simulink model "sm_ratchet_pawl"  (R2025a)
settings: Solver=daessc  StartTime=0.0  StopTime=30  MaxStep=0.01  RelTol=1e-3  AbsTol=1e-3  EnableMultiTasking=on
PreLoadFcn:
  | sm_ratchet_pawl_param
undefined symbols (not defined in the file): A, B, C, D, F, pawl_driver, pawl_locking, ratchet_arm, ratchet_wheel, X, Y, Z
libraries: sm_lib x20, sm_ratchet_pawl_lib x18, nesl_utility x4, fl_lib x3
CloseFcn:
  | try,close(h1_sm_ratchet_pawl),end
  | clear h1_sm_ratchet_pawl
  | try,close(h2_sm_ratchet_pawl),end
  | clear h2_sm_ratchet_pawl
  | try,close(h3_sm_ratchet_pawl),end
  | clear h3_sm_ratchet_pawl
  | try,close(h4_sm_ratchet_pawl),end
  | clear h4_sm_ratchet_pawl
  | 
  | try,close(h1_Extr_Data_Pawl),end
  | try,close(h1_Extr_Data_Ratchet_Wheel),end
Description:
  | Copyright 2024-2026 The MathWorks, Inc.
settings Model: Creator=smiller  LastModifiedBy=smiller
settings SolverCC: AutoScaleAbsTol=off  AlgebraicLoopSolver=TrustRegion  MaxZcPerStep=1.0
settings DataIOCC: LimitDataPoints=on  MaxDataPoints=10000  ReturnWorkspaceOutputs=off  SignalLoggingName=logsout_sm_ratchet_pawl
settings OptimizationCC: ReuseModelBlockBuffer=off  LifeSpan=inf
settings DebuggingCC: UnconnectedInputMsg=warning  UnconnectedOutputMsg=warning  UnconnectedLineMsg=warning  AllowSymbolicDim=off  SubsystemReferenceDiagnosticForUnitTest=warning  SFUnexpectedBacktrackingDiag=warning  SFNoUnconditionalDefaultTransitionDiag=warning  SFExecutionAtInitializationDiag=none  ArithmeticOperatorsInVariantConditions=warning
settings ModelReferenceCC: EnableRefExpFcnMdlSchedulingChecks=on
settings SFSimCC: SimUseLocalCustomCode=off  CustomCodeUndefinedFunction=UseInterfaceOnly
settings RTWCC: RTWUseLocalCustomCode=off  GPUComputeCapability=3.5  DLArmComputeVersion=19.05
settings CodeAppCC: StateflowObjectComments=on
settings GRTTargetCC: TargetLangStandard=C89/C90 (ANSI)
settings ConfigComp: CovMetricSettings=dw  CovSaveCumulativeToWorkspaceVar=on  CovSaveSingleToWorkspaceVar=on  CovExternalEMLEnable=off  CovSFcnEnable=off
settings SimscapeCC: SimscapeLogType=all  SimscapeLogSimulationStatistics=on  SimscapeLogName=simlog_sm_ratchet_pawl  SimscapeLogDataHistory=100000.0
settings ExplorerConfigSet: InternalSimMechanicsExplorerSettings="<ExplorerConfiguration><canonicalview>default</canonicalview><AnimationSetting><BasePlaybackSpeed>1.0</BasePlaybackSpeed><PlaybackSpeedFactor>2.0</PlaybackSpeedFactor></AnimationSetting><TilePanel><TileInfo><Tiles Columns=\"2\" Count=\"3\" Rows=\"2\"><Column Weight=\"0.6446\"/><Column Weight=\"0.3554\"/><Row Weight=\"0.4352\"/><Row Weight=\"0.5648\"/><Tile Height=\"2\" Width=\"1\" X=\"0\" Y=\"0\"/><Tile Height=\"1\" Width=\"1\" X=\"1\" Y=\"0\"/><Tile Height=\"1\" Width=\"1\" X=\"1\" Y=\"1\"/></Tiles></TileInfo><SceneInfo><SceneViewer><BGColor><R>1</R><G>1</G><B>1</B></BGColor><Camera><DoPerspective>off</DoPerspective><Position><X>0.0514746329653971782</X><Y>0.0112521347858783351</Y><Z>0.995249982152964785</Z></Position><Center><X>0.0514746329653971782</X><Y>0.0112521347858783351</Y><Z>-0.00475001784703521501</Z></Center><Up><X>0</X><Y>1</Y><Z>-0</Z></Up><ViewLimDist>1</ViewLimDist><YLim>0.117248588338494303</YLim><XLim>0.158994678564636227</XLim></Camera></SceneViewer><SceneViewer><BGColor><R>1</R><G>1</G><B>1</B></BGColor><Camera><DoPerspective>off</DoPerspective><Position><X>-0.560100967125156224</X><Y>0.346484843060087866</Y><Z>0.771615368247267508</Z></Position><Center><X>-0.00343975445121295865</X><Y>0.095498245923905864</Y><Z>-0.0203025709120879597</Z></Center><Up><X>0.214451241288348721</X><Y>0.964373692155350071</Y><Z>-0.154900119394868807</Z></Up><ViewLimDist>1</ViewLimDist><YLim>0.0292488636148055016</YLim><XLim>0.0509233203174103768</XLim></Camera></SceneViewer><SceneViewer><BGColor><R>1</R><G>1</G><B>1</B></BGColor><Camera><DoPerspective>off</DoPerspective><Position><X>0.849936568602107645</X><Y>0.00451951510809854573</Y><Z>0.588389331993768971</Z></Position><Center><X>0.0650124134104529405</X><Y>0.0227163583315792908</Y><Z>-0.0309352561612741273</Z></Center><Up><X>0.0909807338167105406</X><Y>0.992118625029582368</Y><Z>-0.0861576458800011047</Z></Up><ViewLimDist>1</ViewLimDist><YLim>0.0639705507090228137</YLim><XLim>0.0854896962074708638</XLim></Camera></SceneViewer></SceneInfo></TilePanel><MechEditorPanel><Cameras/><GfxPanelCameraMap/><VideoCreator><PlaybackSpeedRatio>2</PlaybackSpeedRatio><FrameRate>30</FrameRate><VideoFormat>MPEG-4</VideoFormat><FrameSize>auto</FrameSize></VideoCreator></MechEditorPanel></ExplorerConfiguration>"

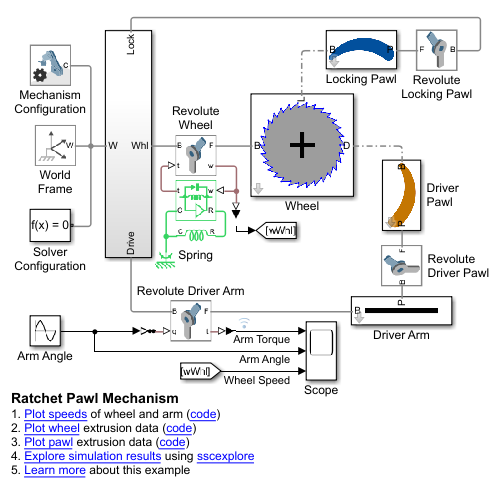
[thumbnail: Simulink's stored preview of the top-level diagram]
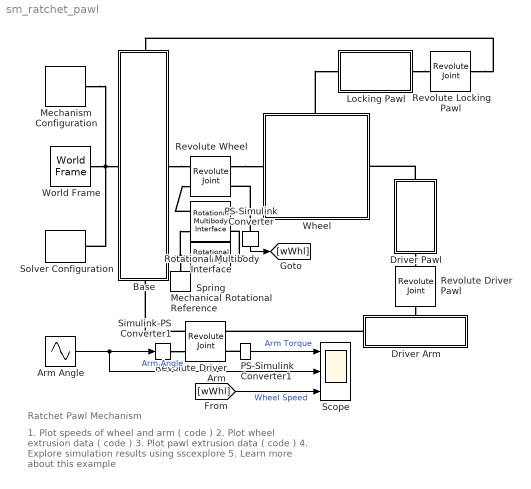
== system sm_ratchet_pawl ==
  note: Ratchet Pawl Mechanism
  note: 1. Plot speeds of wheel and arm ( code )
      | 2. Plot wheel extrusion data ( code )
      | 3. Plot pawl extrusion data ( code )
      | 4. Explore simulation results using sscexplore
      | 5. Learn more about this example
  Arm Angle : Sin  Amplitude=30  Frequency=2*pi/5  SampleTime=0
  Base : Subsystem
      settings: PortSchema="{\"entries\":[{\"content\":{\"sides\":[{\"content\":{\"connectorIds\":[\"LConn1\"]},\"type\":\"ConnectorPlacement.EquallySpacedRectSide\",\"uuid\":\"b6069478-d7cb-4b03-b34f-7e279460368d\"},{\"content\":{\"connectorIds\":[\"RConn1\"],\"side\":\"RIGHT\"},\"type\":\"ConnectorPlacement.EquallySpacedRectSide\",\"uuid\":\"d4387135-640e-415f-ac36-e6f51d44e49d\"},{\"content\":{\"connectorIds\":[\"LConn2\"],\"side\":\"TOP\"},\"type\":\"ConnectorPlacement.EquallySpacedRectSide\",\"uuid\":\"9397bae0-a413-4c70-a9df-3b58371f95bd\"},{\"content\":{\"connectorIds\":[\"RConn2\"],\"side\":\"BOTTOM\"},\"type\":\"ConnectorPlacement.EquallySpacedRectSide\",\"uuid\":\"bb7f362f-dbc7-4f0c-a5eb-cae814777abd\"}]},\"type\":\"ConnectorPlacement.EquallySpacedConnector\",\"uuid\":\"025a31d6-c78e-4390-922c-78c8ee846b7b\"}],\"packageUris\":[\"http://schema.mathworks.com/mf0/Connector/R2020b\"],\"version\":\"1.0\"}"
  Driver Pawl : Subsystem
      mask Display: image('sm_ratchet_pawl_driver_pawl.png');
  Driver Arm : Subsystem
      settings: PortSchema="{\"entries\":[{\"content\":{\"sides\":[{\"content\":{},\"type\":\"ConnectorPlacement.EquallySpacedRectSide\",\"uuid\":\"931ad4cf-5a99-4c9c-9c4c-5cc9ae808209\"},{\"content\":{\"connectorIds\":[\"RConn1\"],\"side\":\"RIGHT\"},\"type\":\"ConnectorPlacement.EquallySpacedRectSide\",\"uuid\":\"6aeb9602-858e-433f-b8ee-b1fa4efa2662\"},{\"content\":{\"connectorIds\":[\"LConn1\"],\"side\":\"TOP\"},\"type\":\"ConnectorPlacement.EquallySpacedRectSide\",\"uuid\":\"8a68191e-bbb5-4d51-a354-3893ab4bb353\"}]},\"type\":\"ConnectorPlacement.EquallySpacedConnector\",\"uuid\":\"f1c0db8b-851d-448f-812d-c20024300439\"}],\"packageUris\":[\"http://schema.mathworks.com/mf0/Connector/R2020b\"],\"version\":\"1.0\"}"
      mask Display: image('sm_ratchet_pawl_driver_arm.png');
  Locking Pawl : Subsystem
      mask Display: image('sm_ratchet_pawl_locking_pawl.png')
  Mechanical Rotational Reference : fl_lib/Mechanical/Rotational Elements/Mechanical Rotational Reference
  Mechanism Configuration : sm_lib/Utilities/Mechanism Configuration  UniformGravity=Constant  GravityVector=[0 0 -9.80665]  GravityVectorUnits=m/s^2  LinearizationDelta=0.001  JointModeTransitionNonlinearIterations=2
  PS-Simulink Converter : nesl_utility/PS-Simulink Converter  PhysicalDomain=network_engine_domain  SubClassName=ps_output  LeftPortType=input  RightPortType=output  PseudoPeriodic=off  Frequencies=[]  VectorFormat=inherit  Unit=inherit  AffineConversion=off
  PS-Simulink Converter1 : nesl_utility/PS-Simulink Converter  PhysicalDomain=network_engine_domain  SubClassName=ps_output  LeftPortType=input  RightPortType=output  PseudoPeriodic=off  Frequencies=[]  VectorFormat=inherit  Unit=1  AffineConversion=off
  Revolute Driver Pawl : sm_lib/Joints/Revolute Joint  JointMode=Normal  CompositeWrenchDir=FollowerOnBase  CompositeWrenchFrame=BaseFrame  SenseConstraintForce=off  SenseConstraintTorque=off  SenseTotalForce=off  SenseTotalTorque=off  PositionTargetSpecify=on  PositionTargetPriority=High  PositionTargetValue=0  PositionTargetValueUnits=deg  VelocityTargetSpecify=off  VelocityTargetPriority=High  VelocityTargetValue=0  VelocityTargetValueUnits=deg/s  EquilibriumPosition=30  EquilibriumPositionUnits=deg  SpringStiffness=0.1  SpringStiffnessUnits=N*m/deg  DampingCoefficient=0.02  DampingCoefficientUnits=N*m/(deg/s)  LowerLimitSpecify=off  LowerLimitBound=-90  LowerLimitBoundUnits=deg  LowerLimitStiffness=1e4  LowerLimitStiffnessUnits=N*m/deg  LowerLimitDamping=10  LowerLimitDampingUnits=N*m/(deg/s)  LowerLimitTransitionRegionWidth=0.1  LowerLimitTransitionRegionWidthUnits=deg  UpperLimitSpecify=off  UpperLimitBound=90  UpperLimitBoundUnits=deg  UpperLimitStiffness=1e4  UpperLimitStiffnessUnits=N*m/deg  UpperLimitDamping=10  UpperLimitDampingUnits=N*m/(deg/s)  UpperLimitTransitionRegionWidth=0.1  UpperLimitTransitionRegionWidthUnits=deg  TorqueActuationMode=NoTorque  MotionActuationMode=ComputedMotion  SensePosition=off  SenseVelocity=off  SenseAcceleration=off  SenseTorqueForce=off  SenseLowerLimitTorqueForce=off  SenseUpperLimitTorqueForce=off
  Revolute Locking Pawl : sm_lib/Joints/Revolute Joint  JointMode=Normal  CompositeWrenchDir=FollowerOnBase  CompositeWrenchFrame=BaseFrame  SenseConstraintForce=off  SenseConstraintTorque=off  SenseTotalForce=off  SenseTotalTorque=off  PositionTargetSpecify=on  PositionTargetPriority=High  PositionTargetValue=90  PositionTargetValueUnits=deg  VelocityTargetSpecify=off  VelocityTargetPriority=High  VelocityTargetValue=0  VelocityTargetValueUnits=deg/s  EquilibriumPosition=110  EquilibriumPositionUnits=deg  SpringStiffness=0.1  SpringStiffnessUnits=N*m/deg  DampingCoefficient=0.02  DampingCoefficientUnits=N*m/(deg/s)  LowerLimitSpecify=off  LowerLimitBound=-90  LowerLimitBoundUnits=deg  LowerLimitStiffness=1e4  LowerLimitStiffnessUnits=N*m/deg  LowerLimitDamping=10  LowerLimitDampingUnits=N*m/(deg/s)  LowerLimitTransitionRegionWidth=0.1  LowerLimitTransitionRegionWidthUnits=deg  UpperLimitSpecify=off  UpperLimitBound=90  UpperLimitBoundUnits=deg  UpperLimitStiffness=1e4  UpperLimitStiffnessUnits=N*m/deg  UpperLimitDamping=10  UpperLimitDampingUnits=N*m/(deg/s)  UpperLimitTransitionRegionWidth=0.1  UpperLimitTransitionRegionWidthUnits=deg  TorqueActuationMode=NoTorque  MotionActuationMode=ComputedMotion  SensePosition=off  SenseVelocity=off  SenseAcceleration=off  SenseTorqueForce=off  SenseLowerLimitTorqueForce=off  SenseUpperLimitTorqueForce=off
  Revolute Wheel : sm_lib/Joints/Revolute Joint  JointMode=Normal  CompositeWrenchDir=FollowerOnBase  CompositeWrenchFrame=BaseFrame  SenseConstraintForce=off  SenseConstraintTorque=off  SenseTotalForce=off  SenseTotalTorque=off  PositionTargetSpecify=off  PositionTargetPriority=High  PositionTargetValue=0  PositionTargetValueUnits=deg  VelocityTargetSpecify=off  VelocityTargetPriority=High  VelocityTargetValue=0  VelocityTargetValueUnits=deg/s  EquilibriumPosition=0  EquilibriumPositionUnits=deg  SpringStiffness=0  SpringStiffnessUnits=N*m/deg  DampingCoefficient=0.1  DampingCoefficientUnits=N*m/(deg/s)  LowerLimitSpecify=off  LowerLimitBound=-90  LowerLimitBoundUnits=deg  LowerLimitStiffness=1e4  LowerLimitStiffnessUnits=N*m/deg  LowerLimitDamping=10  LowerLimitDampingUnits=N*m/(deg/s)  LowerLimitTransitionRegionWidth=0.1  LowerLimitTransitionRegionWidthUnits=deg  UpperLimitSpecify=off  UpperLimitBound=90  UpperLimitBoundUnits=deg  UpperLimitStiffness=1e4  UpperLimitStiffnessUnits=N*m/deg  UpperLimitDamping=10  UpperLimitDampingUnits=N*m/(deg/s)  UpperLimitTransitionRegionWidth=0.1  UpperLimitTransitionRegionWidthUnits=deg  TorqueActuationMode=InputTorque  MotionActuationMode=ComputedMotion  SensePosition=off  SenseVelocity=on  SenseAcceleration=off  SenseTorqueForce=off  SenseLowerLimitTorqueForce=off  SenseUpperLimitTorqueForce=off
  Revolute Driver Arm : sm_lib/Joints/Revolute Joint  JointMode=Normal  CompositeWrenchDir=FollowerOnBase  CompositeWrenchFrame=BaseFrame  SenseConstraintForce=off  SenseConstraintTorque=off  SenseTotalForce=off  SenseTotalTorque=off  PositionTargetSpecify=off  PositionTargetPriority=High  PositionTargetValue=0  PositionTargetValueUnits=deg  VelocityTargetSpecify=off  VelocityTargetPriority=High  VelocityTargetValue=0  VelocityTargetValueUnits=deg/s  EquilibriumPosition=0  EquilibriumPositionUnits=deg  SpringStiffness=0  SpringStiffnessUnits=N*m/deg  DampingCoefficient=0  DampingCoefficientUnits=N*m/(deg/s)  LowerLimitSpecify=off  LowerLimitBound=-90  LowerLimitBoundUnits=deg  LowerLimitStiffness=1e4  LowerLimitStiffnessUnits=N*m/deg  LowerLimitDamping=10  LowerLimitDampingUnits=N*m/(deg/s)  LowerLimitTransitionRegionWidth=0.1  LowerLimitTransitionRegionWidthUnits=deg  UpperLimitSpecify=off  UpperLimitBound=90  UpperLimitBoundUnits=deg  UpperLimitStiffness=1e4  UpperLimitStiffnessUnits=N*m/deg  UpperLimitDamping=10  UpperLimitDampingUnits=N*m/(deg/s)  UpperLimitTransitionRegionWidth=0.1  UpperLimitTransitionRegionWidthUnits=deg  TorqueActuationMode=ComputedTorque  MotionActuationMode=InputMotion  SensePosition=off  SenseVelocity=off  SenseAcceleration=off  SenseTorqueForce=on  SenseLowerLimitTorqueForce=off  SenseUpperLimitTorqueForce=off
  Rotational Multibody Interface : fl_lib/Mechanical/Multibody Interfaces/Rotational Multibody Interface
  Scope : Scope  NumInputPorts=3
      settings: ActiveDisplayYMinimum=-11.66487  ActiveDisplayYMaximum=46.52781
  Simulink-PS Converter1 : nesl_utility/Simulink-PS Converter  PhysicalDomain=network_engine_domain  SubClassName=ps_input  LeftPortType=input  RightPortType=output  PseudoPeriodic=off  Frequencies=[]  NoiseDistribution=none  NoiseParameters=[]  Unit=deg  AffineConversion=off  FilteringAndDerivatives=filter  SimscapeFilterOrder=2  InputFilterTimeConstant=0.1  UdotUserProvided=0
  Solver Configuration : nesl_utility/Solver Configuration  PhysicalDomain=network_engine_domain  SubClassName=solver  LeftPortType=input  RightPortType=generic  Tones=[]  Harmonics=[]  SimulateNoise=off  Profile=off  UseLocalSampling=off  EnableSwitchedLinearOptims=on  FrequencyDomain=off  UseCCode=off  RelTol=0.001  AbsTol=1e-06  MinStep=1e-09  ToWorkspace=off  RevertToSquareIcSolve=off  NumHomotopyIterations=100  PhasorMode=off  PhasorModeNumHarmonics=1  ConsistencySolver=NEWTON_XTOL_AFTER_FTOL  IndexReductionMethod=DerivativeReplacement  DoDC=off  ResidualTolerance=1e-09  ConsistencyTolSource=GLOBAL  ConsistencyAbsTol=0.001  ConsistencyRelTol=0.001  ConsistencyTolFactor=0.001  UseLocalSolver=off  LocalSolverChoice=NE_BACKWARD_EULER_ADVANCER  ResolveIndetEquations=on  FunctionEvalNumThread=1  LocalSolverSampleTime=0.001  DoFixedCost=off  MaxNonlinIter=3  MaxModeIter=2  ComputeImpulses=off  ImpulseIterations=2  LinearAlgebra=Sparse  LinearAlgebraNumThread=0  EquationFormulation=NE_TIME_EF  DelaysMemoryBudget=1024  AutomaticFiltering=on  FilteringTimeConstant=0.001  PartitionStorageMethod=AS_NEEDED  PartitionMemoryBudget=1024  PartitionMethod=FAST  MultibodyUseLocalSolver=off  MultibodyLocalSolverChoice=ODE1  MultibodyLocalSolverSampleTime=0.001
  Spring : fl_lib/Mechanical/Rotational Elements/Rotational Spring  spr_rate=10 N*m/rad  w_specify=off  w_priority=None  w=0 rad/s  w_nominal_specify=off  w_nominal_value=1  w_nominal_unit=rad/s  t_specify=off  t_priority=None  t=0 N*m  t_nominal_specify=off  t_nominal_value=1  t_nominal_unit=N*m  phi_specify=off  phi_priority=High  phi=0 rad  phi_nominal_specify=off  phi_nominal_value=1  phi_nominal_unit=rad
  Wheel : Subsystem
      settings: PortSchema="{\"entries\":[{\"content\":{\"sides\":[{\"content\":{\"connectorIds\":[\"LConn1\"]},\"type\":\"ConnectorPlacement.EquallySpacedRectSide\",\"uuid\":\"04441881-9c30-4d5d-be6a-59ca06764360\"},{\"content\":{\"connectorIds\":[\"RConn1\"],\"side\":\"RIGHT\"},\"type\":\"ConnectorPlacement.EquallySpacedRectSide\",\"uuid\":\"fa22e8ef-2b3e-4a8e-b49c-1688172feace\"},{\"content\":{\"connectorIds\":[\"LConn2\"],\"side\":\"TOP\"},\"type\":\"ConnectorPlacement.EquallySpacedRectSide\",\"uuid\":\"207ec217-ed21-440a-9842-994c4e25d04a\"}]},\"type\":\"ConnectorPlacement.EquallySpacedConnector\",\"uuid\":\"e84f3840-6153-4aef-b387-4bc57ec5edf1\"}],\"packageUris\":[\"http://schema.mathworks.com/mf0/Connector/R2020b\"],\"version\":\"1.0\"}"
      mask Display: image('sm_ratchet_pawl_wheel_lines.png')
  World Frame : sm_lib/Frames and Transforms/World Frame
  wires:
  [wWhl] -> Scope/3  "Wheel Speed"
  Arm Angle/1 -> Simulink-PS Converter1/1, Scope/2  "Arm Angle"
  PS-Simulink Converter1/1 -> Scope/1  "Arm Torque"
  PS-Simulink Converter/1 -> [wWhl]
  connections:
  World Frame/RConn1 -- Solver Configuration/RConn1 -- Base/LConn1 -- Mechanism Configuration/RConn1
  Driver Arm/RConn1 -- Revolute Driver Arm/RConn1
  Revolute Driver Pawl/LConn1 -- Driver Arm/LConn1
  Driver Pawl/RConn1 -- Revolute Driver Pawl/RConn1
  Revolute Wheel/RConn1 -- Wheel/LConn1
  Driver Pawl/LConn1 -- Wheel/RConn1
  Locking Pawl/RConn1 -- Revolute Locking Pawl/RConn1
  Wheel/LConn2 -- Locking Pawl/LConn1
  Simulink-PS Converter1/RConn1 -- Revolute Driver Arm/LConn2
  Revolute Locking Pawl/LConn1 -- Base/LConn2
  Revolute Driver Arm/LConn1 -- Base/RConn2
  Base/RConn1 -- Revolute Wheel/LConn1
  PS-Simulink Converter1/LConn1 -- Revolute Driver Arm/RConn2
  PS-Simulink Converter/LConn1 -- Rotational Multibody Interface/RConn1 -- Revolute Wheel/RConn2
  Rotational Multibody Interface/LConn1 -- Revolute Wheel/LConn2
  Spring/LConn1 -- Rotational Multibody Interface/RConn2
  Spring/RConn1 -- Mechanical Rotational Reference/LConn1 -- Rotational Multibody Interface/LConn2

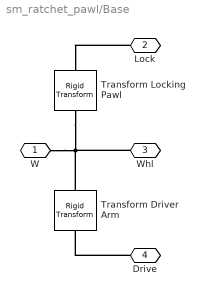
== system sm_ratchet_pawl/Base ==
  Transform Driver Arm : sm_lib/Frames and Transforms/Rigid Transform  RotationMethod=None  FollAlignAxisA=+X  BaseAlignAxisA=+Y  FollAlignAxisB=+Y  BaseAlignAxisB=+Z  RotationStandardAxis=+Z  RotationAngle=0.0  RotationAngleUnits=deg  RotationArbitraryAxis=[0 0 1]  RotationSequenceAxes=FollowerAxes  RotationSequence=XYX  RotationSequenceAngles=[0 0 0]  RotationSequenceAnglesUnits=deg  RotationMatrix=[1 0 0; 0 1 0; 0 0 1]  Quaternion=[1 0 0 0]  TranslationMethod=StandardAxis  TranslationCartesianOffset=[0 0 0]  TranslationCartesianOffsetUnits=m  TranslationStandardAxis=+Z  TranslationStandardOffset=-(ratchet_arm.depth+ratchet_wheel.depth)/2  TranslationStandardOffsetUnits=m  TranslationROffset=0  TranslationROffsetUnits=m  TranslationThetaOffset=0  TranslationThetaOffsetUnits=deg  TranslationZOffset=0  TranslationZOffsetUnits=m
  Transform Locking Pawl : sm_lib/Frames and Transforms/Rigid Transform  RotationMethod=None  FollAlignAxisA=+X  BaseAlignAxisA=+Y  FollAlignAxisB=+Y  BaseAlignAxisB=+Z  RotationStandardAxis=+Z  RotationAngle=0.0  RotationAngleUnits=deg  RotationArbitraryAxis=[0 0 1]  RotationSequenceAxes=FollowerAxes  RotationSequence=XYX  RotationSequenceAngles=[0 0 0]  RotationSequenceAnglesUnits=deg  RotationMatrix=[1 0 0; 0 1 0; 0 0 1]  Quaternion=[1 0 0 0]  TranslationMethod=Cartesian  TranslationCartesianOffset=[0 pawl_locking.offset -ratchet_wheel.depth/2]  TranslationCartesianOffsetUnits=m  TranslationStandardAxis=+Y  TranslationStandardOffset=0.15  TranslationStandardOffsetUnits=m  TranslationROffset=0  TranslationROffsetUnits=m  TranslationThetaOffset=0  TranslationThetaOffsetUnits=deg  TranslationZOffset=0  TranslationZOffsetUnits=m
  W : PMIOPort  Side=Left
  Lock : PMIOPort  Port=2  Side=Left
  Whl : PMIOPort  Port=3  Side=Right
  Drive : PMIOPort  Port=4  Side=Right
  connections:
  Drive/RConn1 -- Transform Driver Arm/RConn1
  Lock/RConn1 -- Transform Locking Pawl/RConn1
  W/RConn1 -- Whl/RConn1 -- Transform Driver Arm/LConn1 -- Transform Locking Pawl/LConn1

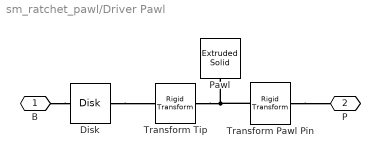
== system sm_ratchet_pawl/Driver Pawl ==
  Disk : sm_lib/Curves and Surfaces/Disk  Radius=pawl_driver.tip_rad  RadiusUnits=m  GraphicType=FromGeometry  GraphicVisPropType=SimpleVisualProperties  GraphicDiffuseColor=[0 0 1]  GraphicOpacity=1.0  GraphicSpecularColor=[0.5 0.5 0.5 1.0]  GraphicAmbientColor=[0.15 0.15 0.15 1.0]  GraphicEmissiveColor=[0.0 0.0 0.0 1.0]  GraphicShininess=75
  Pawl : sm_lib/Body Elements/Extruded Solid  ExtrusionType=General  PolygonNumSides=3  PolygonOuterRadius=1  PolygonOuterRadiusUnits=m  ExportEntireGeometry=off  ExtrusionCrossSection=pawl_driver.xsect  ExtrusionCrossSectionUnits=m  ExportConvexHullGeometry=off  ExtrusionLength=0.01  ExtrusionLengthUnits=m  InertiaType=CalculateFromGeometry  BasedOnType=Density  Density=1000  DensityUnits=kg/m^3  Mass=1  MassUnits=kg  CenterOfMass=[0 0 0]  CenterOfMassUnits=m  MomentsOfInertia=[1 1 1]  MomentsOfInertiaUnits=kg*m^2  ProductsOfInertia=[0 0 0]  ProductsOfInertiaUnits=kg*m^2  GraphicType=FromGeometry  MarkerShape=Sphere  MarkerSize=10  GraphicVisPropType=SimpleVisualProperties  GraphicDiffuseColor=[1.0 0.6 0.0]  GraphicOpacity=1.0  GraphicSpecularColor=[0.5 0.5 0.5 1.0]  GraphicAmbientColor=[0.15 0.15 0.15 1.0]  GraphicEmissiveColor=[0.0 0.0 0.0 1.0]  GraphicShininess=75  DoExposeReferenceFrame=on  SerializedFrames=<Frames/>
  Transform Pawl Pin : sm_lib/Frames and Transforms/Rigid Transform  RotationMethod=None  FollAlignAxisA=+X  BaseAlignAxisA=+Y  FollAlignAxisB=+Y  BaseAlignAxisB=+Z  RotationStandardAxis=+Z  RotationAngle=0.0  RotationAngleUnits=deg  RotationArbitraryAxis=[0 0 1]  RotationSequenceAxes=FollowerAxes  RotationSequence=XYX  RotationSequenceAngles=[0 0 0]  RotationSequenceAnglesUnits=deg  RotationMatrix=[1 0 0; 0 1 0; 0 0 1]  Quaternion=[1 0 0 0]  TranslationMethod=StandardAxis  TranslationCartesianOffset=[0 0 0]  TranslationCartesianOffsetUnits=m  TranslationStandardAxis=+Z  TranslationStandardOffset=-0.005  TranslationStandardOffsetUnits=m  TranslationROffset=0  TranslationROffsetUnits=m  TranslationThetaOffset=0  TranslationThetaOffsetUnits=deg  TranslationZOffset=0  TranslationZOffsetUnits=m
  Transform Tip : sm_lib/Frames and Transforms/Rigid Transform  RotationMethod=None  FollAlignAxisA=+X  BaseAlignAxisA=+Y  FollAlignAxisB=+Y  BaseAlignAxisB=+Z  RotationStandardAxis=+Z  RotationAngle=0.0  RotationAngleUnits=deg  RotationArbitraryAxis=[0 0 1]  RotationSequenceAxes=FollowerAxes  RotationSequence=XYX  RotationSequenceAngles=[0 0 0]  RotationSequenceAnglesUnits=deg  RotationMatrix=[1 0 0; 0 1 0; 0 0 1]  Quaternion=[1 0 0 0]  TranslationMethod=Cartesian  TranslationCartesianOffset=[pawl_driver.cFrame(1,1) pawl_driver.cFrame(1,2) 0]  TranslationCartesianOffsetUnits=m  TranslationStandardAxis=+Z  TranslationStandardOffset=0  TranslationStandardOffsetUnits=m  TranslationROffset=0  TranslationROffsetUnits=m  TranslationThetaOffset=0  TranslationThetaOffsetUnits=deg  TranslationZOffset=0  TranslationZOffsetUnits=m
  B : PMIOPort  Side=Left
  P : PMIOPort  Port=2  Side=Right
  connections:
  Transform Pawl Pin/RConn1 -- P/RConn1
  Transform Pawl Pin/LConn1 -- Transform Tip/LConn1 -- Pawl/RConn1
  Disk/LConn1 -- Transform Tip/RConn1
  B/RConn1 -- Disk/RConn1

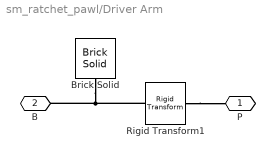
== system sm_ratchet_pawl/Driver Arm ==
  Brick Solid : sm_lib/Body Elements/Brick Solid  BrickDimensions=[ratchet_arm. length ratchet_arm.depth ratchet_arm.depth]  BrickDimensionsUnits=m  ExportEntireGeometry=off  InertiaType=CalculateFromGeometry  BasedOnType=Density  Density=1000  DensityUnits=kg/m^3  Mass=1  MassUnits=kg  CenterOfMass=[0 0 0]  CenterOfMassUnits=m  MomentsOfInertia=[1 1 1]  MomentsOfInertiaUnits=kg*m^2  ProductsOfInertia=[0 0 0]  ProductsOfInertiaUnits=kg*m^2  GraphicType=FromGeometry  MarkerShape=Sphere  MarkerSize=10  GraphicVisPropType=SimpleVisualProperties  GraphicDiffuseColor=[0.0 0.0 0.0]  GraphicOpacity=1.0  GraphicSpecularColor=[0.5 0.5 0.5 1.0]  GraphicAmbientColor=[0.15 0.15 0.15 1.0]  GraphicEmissiveColor=[0.0 0.0 0.0 1.0]  GraphicShininess=75  DoExposeReferenceFrame=off  SerializedFrames=<Frames><Frame><Id>Frame1</Id><Value><Name>B</Name><Origin><Source>GeometricFeature</Source><FeatureName>-x surface</FeatureName></Origin><PrimaryAxis><DefinedDirection>+Z</DefinedDirection><Source>ReferenceFrame</Source><SourceDirection>+Z</SourceDirection><FeatureName></FeatureName></PrimaryAxis><SecondaryAxis><DefinedDirection>+X</DefinedDirection><Source>ReferenceFrame</Source><SourceDirection>+X</SourceDirection><FeatureName></FeatureName></SecondaryAxis></Value></Frame></Frames>
  Rigid Transform1 : sm_lib/Frames and Transforms/Rigid Transform  RotationMethod=None  FollAlignAxisA=+X  BaseAlignAxisA=+Y  FollAlignAxisB=+Y  BaseAlignAxisB=+Z  RotationStandardAxis=+Z  RotationAngle=0.0  RotationAngleUnits=deg  RotationArbitraryAxis=[0 0 1]  RotationSequenceAxes=FollowerAxes  RotationSequence=XYX  RotationSequenceAngles=[0 0 0]  RotationSequenceAnglesUnits=deg  RotationMatrix=[1 0 0; 0 1 0; 0 0 1]  Quaternion=[1 0 0 0]  TranslationMethod=Cartesian  TranslationCartesianOffset=[pawl_driver.offset 0 ratchet_arm.depth/2]  TranslationCartesianOffsetUnits=m  TranslationStandardAxis=+X  TranslationStandardOffset=0.15  TranslationStandardOffsetUnits=m  TranslationROffset=0  TranslationROffsetUnits=m  TranslationThetaOffset=0  TranslationThetaOffsetUnits=deg  TranslationZOffset=0  TranslationZOffsetUnits=m
  P : PMIOPort  Side=Left
  B : PMIOPort  Port=2  Side=Right
  connections:
  Brick Solid/LConn1 -- Rigid Transform1/LConn1 -- B/RConn1
  Rigid Transform1/RConn1 -- P/RConn1

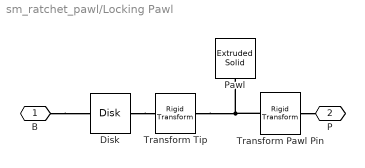
== system sm_ratchet_pawl/Locking Pawl ==
  Disk : sm_lib/Curves and Surfaces/Disk  Radius=pawl_locking.tip_rad  RadiusUnits=m  GraphicType=FromGeometry  GraphicVisPropType=SimpleVisualProperties  GraphicDiffuseColor=[0 0 1]  GraphicOpacity=1.0  GraphicSpecularColor=[0.5 0.5 0.5 1.0]  GraphicAmbientColor=[0.15 0.15 0.15 1.0]  GraphicEmissiveColor=[0.0 0.0 0.0 1.0]  GraphicShininess=75
  Pawl : sm_lib/Body Elements/Extruded Solid  ExtrusionType=General  PolygonNumSides=3  PolygonOuterRadius=1  PolygonOuterRadiusUnits=m  ExportEntireGeometry=off  ExtrusionCrossSection=pawl_locking.xsect  ExtrusionCrossSectionUnits=m  ExportConvexHullGeometry=off  ExtrusionLength=0.01  ExtrusionLengthUnits=m  InertiaType=CalculateFromGeometry  BasedOnType=Density  Density=1000  DensityUnits=kg/m^3  Mass=1  MassUnits=kg  CenterOfMass=[0 0 0]  CenterOfMassUnits=m  MomentsOfInertia=[1 1 1]  MomentsOfInertiaUnits=kg*m^2  ProductsOfInertia=[0 0 0]  ProductsOfInertiaUnits=kg*m^2  GraphicType=FromGeometry  MarkerShape=Sphere  MarkerSize=10  GraphicVisPropType=SimpleVisualProperties  GraphicDiffuseColor=[0.0 0.4 0.8]  GraphicOpacity=1.0  GraphicSpecularColor=[0.5 0.5 0.5 1.0]  GraphicAmbientColor=[0.15 0.15 0.15 1.0]  GraphicEmissiveColor=[0.0 0.0 0.0 1.0]  GraphicShininess=75  DoExposeReferenceFrame=on  SerializedFrames=<Frames/>
  Transform Pawl Pin : sm_lib/Frames and Transforms/Rigid Transform  RotationMethod=None  FollAlignAxisA=+X  BaseAlignAxisA=+Y  FollAlignAxisB=+Y  BaseAlignAxisB=+Z  RotationStandardAxis=+Z  RotationAngle=0.0  RotationAngleUnits=deg  RotationArbitraryAxis=[0 0 1]  RotationSequenceAxes=FollowerAxes  RotationSequence=XYX  RotationSequenceAngles=[0 0 0]  RotationSequenceAnglesUnits=deg  RotationMatrix=[1 0 0; 0 1 0; 0 0 1]  Quaternion=[1 0 0 0]  TranslationMethod=StandardAxis  TranslationCartesianOffset=[0 0 0]  TranslationCartesianOffsetUnits=m  TranslationStandardAxis=+Z  TranslationStandardOffset=-0.005  TranslationStandardOffsetUnits=m  TranslationROffset=0  TranslationROffsetUnits=m  TranslationThetaOffset=0  TranslationThetaOffsetUnits=deg  TranslationZOffset=0  TranslationZOffsetUnits=m
  Transform Tip : sm_lib/Frames and Transforms/Rigid Transform  RotationMethod=None  FollAlignAxisA=+X  BaseAlignAxisA=+Y  FollAlignAxisB=+Y  BaseAlignAxisB=+Z  RotationStandardAxis=+Z  RotationAngle=0.0  RotationAngleUnits=deg  RotationArbitraryAxis=[0 0 1]  RotationSequenceAxes=FollowerAxes  RotationSequence=XYX  RotationSequenceAngles=[0 0 0]  RotationSequenceAnglesUnits=deg  RotationMatrix=[1 0 0; 0 1 0; 0 0 1]  Quaternion=[1 0 0 0]  TranslationMethod=Cartesian  TranslationCartesianOffset=[pawl_locking.cFrame(1,1) pawl_locking.cFrame(1,2) 0]  TranslationCartesianOffsetUnits=m  TranslationStandardAxis=+Z  TranslationStandardOffset=0  TranslationStandardOffsetUnits=m  TranslationROffset=0  TranslationROffsetUnits=m  TranslationThetaOffset=0  TranslationThetaOffsetUnits=deg  TranslationZOffset=0  TranslationZOffsetUnits=m
  B : PMIOPort  Side=Left
  P : PMIOPort  Port=2  Side=Right
  connections:
  B/RConn1 -- Disk/RConn1
  Disk/LConn1 -- Transform Tip/RConn1
  Transform Tip/LConn1 -- Transform Pawl Pin/LConn1 -- Pawl/RConn1
  Transform Pawl Pin/RConn1 -- P/RConn1

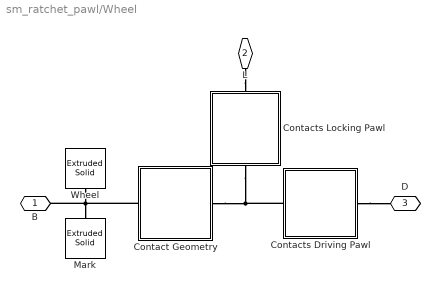
== system sm_ratchet_pawl/Wheel ==
  Contact Geometry : Subsystem
      mask Display: image('sm_ratchet_pawl_lines.png')
  Contacts Driving Pawl : Subsystem
  Contacts Locking Pawl : Subsystem
  Mark : sm_lib/Body Elements/Extruded Solid  ExtrusionType=General  PolygonNumSides=6  PolygonOuterRadius=0.02  PolygonOuterRadiusUnits=m  ExportEntireGeometry=off  ExtrusionCrossSection=[1 1; 1 6; -1 6; -1 1; -6 1; -6 -1; -1 -1; -1 -6; 1 -6; 1 -1; 6 -1; 6 1]*0.005  ExtrusionCrossSectionUnits=m  ExportConvexHullGeometry=off  ExtrusionLength=0.011  ExtrusionLengthUnits=m  InertiaType=CalculateFromGeometry  BasedOnType=Density  Density=1000  DensityUnits=kg/m^3  Mass=1  MassUnits=kg  CenterOfMass=[0 0 0]  CenterOfMassUnits=m  MomentsOfInertia=[1 1 1]  MomentsOfInertiaUnits=kg*m^2  ProductsOfInertia=[0 0 0]  ProductsOfInertiaUnits=kg*m^2  GraphicType=FromGeometry  MarkerShape=Sphere  MarkerSize=10  GraphicVisPropType=SimpleVisualProperties  GraphicDiffuseColor=[0.0 0.0 0.0]  GraphicOpacity=1.0  GraphicSpecularColor=[0.5 0.5 0.5 1.0]  GraphicAmbientColor=[0.15 0.15 0.15 1.0]  GraphicEmissiveColor=[0.0 0.0 0.0 1.0]  GraphicShininess=75  DoExposeReferenceFrame=on  SerializedFrames=<Frames/>
  Wheel : sm_lib/Body Elements/Extruded Solid  ExtrusionType=General  PolygonNumSides=3  PolygonOuterRadius=1  PolygonOuterRadiusUnits=m  ExportEntireGeometry=off  ExtrusionCrossSection=ratchet_wheel.xsect  ExtrusionCrossSectionUnits=m  ExportConvexHullGeometry=off  ExtrusionLength=ratchet_wheel.depth  ExtrusionLengthUnits=m  InertiaType=CalculateFromGeometry  BasedOnType=Density  Density=1000  DensityUnits=kg/m^3  Mass=1  MassUnits=kg  CenterOfMass=[0 0 0]  CenterOfMassUnits=m  MomentsOfInertia=[1 1 1]  MomentsOfInertiaUnits=kg*m^2  ProductsOfInertia=[0 0 0]  ProductsOfInertiaUnits=kg*m^2  GraphicType=FromGeometry  MarkerShape=Sphere  MarkerSize=10  GraphicVisPropType=SimpleVisualProperties  GraphicDiffuseColor=[0.8 0.8 0.8]  GraphicOpacity=1.0  GraphicSpecularColor=[0.5 0.5 0.5 1.0]  GraphicAmbientColor=[0.15 0.15 0.15 1.0]  GraphicEmissiveColor=[0.0 0.0 0.0 1.0]  GraphicShininess=75  DoExposeReferenceFrame=on  SerializedFrames=<Frames/>
  B : PMIOPort  Side=Left
  L : PMIOPort  Port=2  Side=Left
  D : PMIOPort  Port=3  Side=Right
  connections:
  Contacts Locking Pawl/LConn1 -- Contacts Driving Pawl/LConn1 -- Contact Geometry/RConn1
  L/RConn1 -- Contacts Locking Pawl/RConn1
  Contacts Driving Pawl/RConn1 -- D/RConn1
  Wheel/RConn1 -- Contact Geometry/LConn1 -- B/RConn1 -- Mark/RConn1

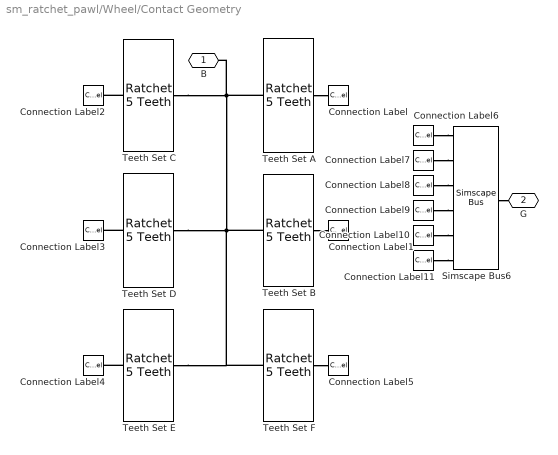
== system sm_ratchet_pawl/Wheel/Contact Geometry ==
  Connection Label : ConnectionLabel  Label=A
  Connection Label1 : ConnectionLabel  Label=B
  Connection Label10 : ConnectionLabel  Label=E
  Connection Label11 : ConnectionLabel  Label=F
  Connection Label2 : ConnectionLabel  Label=C
  Connection Label3 : ConnectionLabel  Label=D
  Connection Label4 : ConnectionLabel  Label=E
  Connection Label5 : ConnectionLabel  Label=F
  Connection Label6 : ConnectionLabel  Label=A
  Connection Label7 : ConnectionLabel  Label=B
  Connection Label8 : ConnectionLabel  Label=C
  Connection Label9 : ConnectionLabel  Label=D
  Simscape Bus6 : SimscapeBus  HierarchyStrings=A;B;C;D;E;F
  Teeth Set A : sm_ratchet_pawl_lib/Ratchet 5 Teeth  ind_set=0
  Teeth Set B : sm_ratchet_pawl_lib/Ratchet 5 Teeth  ind_set=10
  Teeth Set C : sm_ratchet_pawl_lib/Ratchet 5 Teeth  ind_set=20
  Teeth Set D : sm_ratchet_pawl_lib/Ratchet 5 Teeth  ind_set=30
  Teeth Set E : sm_ratchet_pawl_lib/Ratchet 5 Teeth  ind_set=40
  Teeth Set F : sm_ratchet_pawl_lib/Ratchet 5 Teeth  ind_set=50
  B : PMIOPort  Side=Left
  G : PMIOPort  Port=2  Side=Right
  connections:
  Teeth Set C/LConn1 -- Teeth Set B/LConn1 -- Teeth Set F/LConn1 -- Teeth Set E/LConn1 -- Teeth Set D/LConn1 -- Teeth Set A/LConn1 -- B/RConn1
  Connection Label10/LConn1 -- Simscape Bus6/LConn5
  Teeth Set E/RConn1 -- Connection Label4/LConn1
  Connection Label9/LConn1 -- Simscape Bus6/LConn4
  Simscape Bus6/RConn1 -- G/RConn1
  Teeth Set C/RConn1 -- Connection Label2/LConn1
  Teeth Set F/RConn1 -- Connection Label5/LConn1
  Teeth Set B/RConn1 -- Connection Label1/LConn1
  Connection Label7/LConn1 -- Simscape Bus6/LConn2
  Connection Label6/LConn1 -- Simscape Bus6/LConn1
  Teeth Set D/RConn1 -- Connection Label3/LConn1
  Connection Label11/LConn1 -- Simscape Bus6/LConn6
  Connection Label8/LConn1 -- Simscape Bus6/LConn3
  Teeth Set A/RConn1 -- Connection Label/LConn1

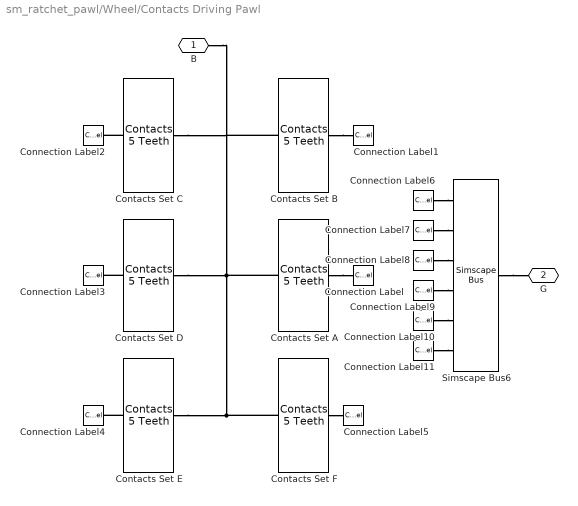
== system sm_ratchet_pawl/Wheel/Contacts Driving Pawl ==
  Connection Label : ConnectionLabel  Label=A
  Connection Label1 : ConnectionLabel  Label=B
  Connection Label10 : ConnectionLabel  Label=E
  Connection Label11 : ConnectionLabel  Label=F
  Connection Label2 : ConnectionLabel  Label=C
  Connection Label3 : ConnectionLabel  Label=D
  Connection Label4 : ConnectionLabel  Label=E
  Connection Label5 : ConnectionLabel  Label=F
  Connection Label6 : ConnectionLabel  Label=A
  Connection Label7 : ConnectionLabel  Label=B
  Connection Label8 : ConnectionLabel  Label=C
  Connection Label9 : ConnectionLabel  Label=D
  Contacts Set A : sm_ratchet_pawl_lib/Contacts 5 Teeth  k_whl=contact_WR.k  b_whl=contact_WR.b  x_whl=contact_WR.x  s_whl=contact_WR.s  d_whl=contact_WR.d  v_whl=contact_WR.v
  Contacts Set B : sm_ratchet_pawl_lib/Contacts 5 Teeth  k_whl=contact_WR.k  b_whl=contact_WR.b  x_whl=contact_WR.x  s_whl=contact_WR.s  d_whl=contact_WR.d  v_whl=contact_WR.v
  Contacts Set C : sm_ratchet_pawl_lib/Contacts 5 Teeth  k_whl=contact_WR.k  b_whl=contact_WR.b  x_whl=contact_WR.x  s_whl=contact_WR.s  d_whl=contact_WR.d  v_whl=contact_WR.v
  Contacts Set D : sm_ratchet_pawl_lib/Contacts 5 Teeth  k_whl=contact_WR.k  b_whl=contact_WR.b  x_whl=contact_WR.x  s_whl=contact_WR.s  d_whl=contact_WR.d  v_whl=contact_WR.v
  Contacts Set E : sm_ratchet_pawl_lib/Contacts 5 Teeth  k_whl=contact_WR.k  b_whl=contact_WR.b  x_whl=contact_WR.x  s_whl=contact_WR.s  d_whl=contact_WR.d  v_whl=contact_WR.v
  Contacts Set F : sm_ratchet_pawl_lib/Contacts 5 Teeth  k_whl=contact_WR.k  b_whl=contact_WR.b  x_whl=contact_WR.x  s_whl=contact_WR.s  d_whl=contact_WR.d  v_whl=contact_WR.v
  Simscape Bus6 : SimscapeBus  HierarchyStrings=A;B;C;D;E;F
  B : PMIOPort  Side=Right
  G : PMIOPort  Port=2  Side=Left
  connections:
  Simscape Bus6/RConn1 -- G/RConn1
  Contacts Set A/RConn1 -- Connection Label/LConn1
  Contacts Set D/RConn1 -- Connection Label3/LConn1
  Connection Label8/LConn1 -- Simscape Bus6/LConn3
  Contacts Set E/RConn1 -- Connection Label4/LConn1
  Contacts Set C/RConn1 -- Connection Label2/LConn1
  Connection Label11/LConn1 -- Simscape Bus6/LConn6
  Connection Label6/LConn1 -- Simscape Bus6/LConn1
  Connection Label7/LConn1 -- Simscape Bus6/LConn2
  Connection Label10/LConn1 -- Simscape Bus6/LConn5
  Connection Label9/LConn1 -- Simscape Bus6/LConn4
  Contacts Set A/LConn1 -- Contacts Set D/LConn1 -- B/RConn1 -- Contacts Set B/LConn1 -- Contacts Set C/LConn1 -- Contacts Set E/LConn1 -- Contacts Set F/LConn1
  Contacts Set F/RConn1 -- Connection Label5/LConn1
  Contacts Set B/RConn1 -- Connection Label1/LConn1

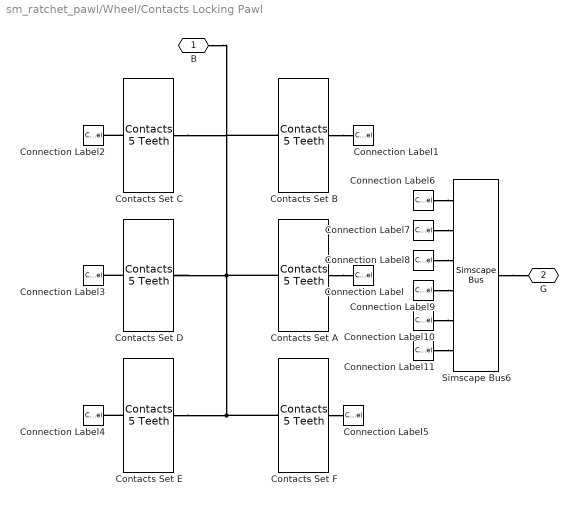
== system sm_ratchet_pawl/Wheel/Contacts Locking Pawl ==
  Connection Label : ConnectionLabel  Label=A
  Connection Label1 : ConnectionLabel  Label=B
  Connection Label10 : ConnectionLabel  Label=E
  Connection Label11 : ConnectionLabel  Label=F
  Connection Label2 : ConnectionLabel  Label=C
  Connection Label3 : ConnectionLabel  Label=D
  Connection Label4 : ConnectionLabel  Label=E
  Connection Label5 : ConnectionLabel  Label=F
  Connection Label6 : ConnectionLabel  Label=A
  Connection Label7 : ConnectionLabel  Label=B
  Connection Label8 : ConnectionLabel  Label=C
  Connection Label9 : ConnectionLabel  Label=D
  Contacts Set A : sm_ratchet_pawl_lib/Contacts 5 Teeth  k_whl=contact_WR.k  b_whl=contact_WR.b  x_whl=contact_WR.x  s_whl=contact_WR.s  d_whl=contact_WR.d  v_whl=contact_WR.v
  Contacts Set B : sm_ratchet_pawl_lib/Contacts 5 Teeth  k_whl=contact_WR.k  b_whl=contact_WR.b  x_whl=contact_WR.x  s_whl=contact_WR.s  d_whl=contact_WR.d  v_whl=contact_WR.v
  Contacts Set C : sm_ratchet_pawl_lib/Contacts 5 Teeth  k_whl=contact_WR.k  b_whl=contact_WR.b  x_whl=contact_WR.x  s_whl=contact_WR.s  d_whl=contact_WR.d  v_whl=contact_WR.v
  Contacts Set D : sm_ratchet_pawl_lib/Contacts 5 Teeth  k_whl=contact_WR.k  b_whl=contact_WR.b  x_whl=contact_WR.x  s_whl=contact_WR.s  d_whl=contact_WR.d  v_whl=contact_WR.v
  Contacts Set E : sm_ratchet_pawl_lib/Contacts 5 Teeth  k_whl=contact_WR.k  b_whl=contact_WR.b  x_whl=contact_WR.x  s_whl=contact_WR.s  d_whl=contact_WR.d  v_whl=contact_WR.v
  Contacts Set F : sm_ratchet_pawl_lib/Contacts 5 Teeth  k_whl=contact_WR.k  b_whl=contact_WR.b  x_whl=contact_WR.x  s_whl=contact_WR.s  d_whl=contact_WR.d  v_whl=contact_WR.v
  Simscape Bus6 : SimscapeBus  HierarchyStrings=A;B;C;D;E;F
  B : PMIOPort  Side=Right
  G : PMIOPort  Port=2  Side=Left
  connections:
  Contacts Set B/RConn1 -- Connection Label1/LConn1
  Contacts Set F/RConn1 -- Connection Label5/LConn1
  Contacts Set C/LConn1 -- Contacts Set B/LConn1 -- B/RConn1 -- Contacts Set F/LConn1 -- Contacts Set E/LConn1 -- Contacts Set D/LConn1 -- Contacts Set A/LConn1
  Connection Label9/LConn1 -- Simscape Bus6/LConn4
  Connection Label10/LConn1 -- Simscape Bus6/LConn5
  Connection Label7/LConn1 -- Simscape Bus6/LConn2
  Connection Label6/LConn1 -- Simscape Bus6/LConn1
  Connection Label11/LConn1 -- Simscape Bus6/LConn6
  Contacts Set C/RConn1 -- Connection Label2/LConn1
  Contacts Set E/RConn1 -- Connection Label4/LConn1
  Connection Label8/LConn1 -- Simscape Bus6/LConn3
  Contacts Set D/RConn1 -- Connection Label3/LConn1
  Contacts Set A/RConn1 -- Connection Label/LConn1
  Simscape Bus6/RConn1 -- G/RConn1
